simulink model "Roll_Pitch_Mixer_Disturbance_Baseline"  (R2026b)
settings: Solver=FixedStepDiscrete  StopTime=15  FixedStep=0.01
model workspace (MAT data in the model file):
  K_achieved = [1  1  1  1; -0.0742462128401  -0.0742462128401  0.0742462128401  0.0742462128401; -0.0742462128401  0.0742462128401  -0.0742462128401  0.0742462128401]
  d_arm = 0.0742462128401
undefined symbols (not defined in the file): DiscIntNeverNeededParam

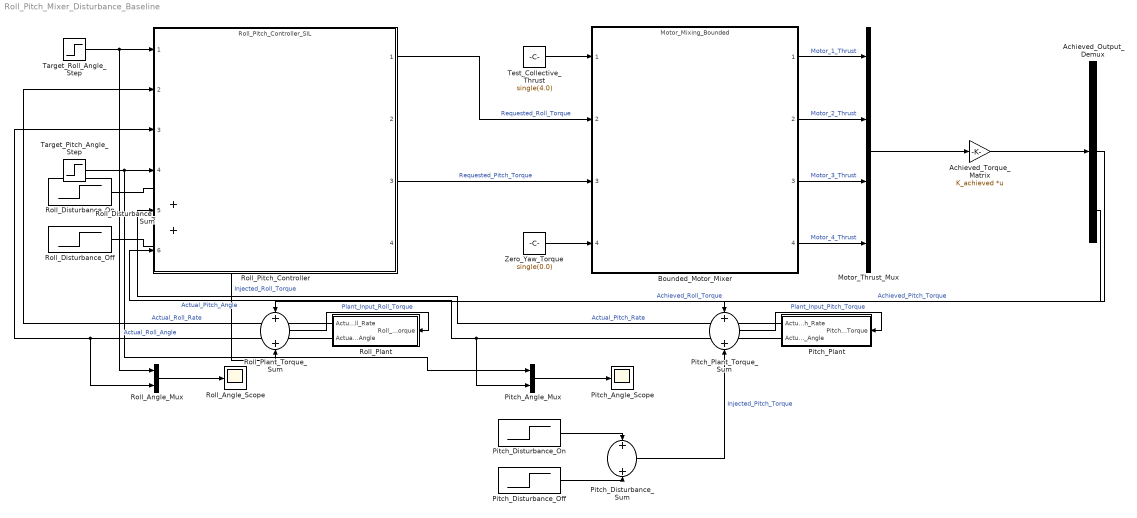
== system Roll_Pitch_Mixer_Disturbance_Baseline ==
  Achieved_Output_Demux : Demux  Outputs=3
  Achieved_Torque_Matrix : Gain  Gain=K_achieved  Multiplication=Matrix(K*u)
  Bounded_Motor_Mixer : ModelReference  ModelNameDialog=Motor_Mixing_Bounded  SimulationMode=Normal  ModelReferenceVersion=1.9
  Motor_Thrust_Mux : Mux
  Pitch_Angle_Mux : Mux  Inputs=2
  Pitch_Angle_Scope : Scope
      settings: ActiveDisplayYMinimum=-0.0589651926420629  ActiveDisplayYMaximum=0.0065516880713403208
  Pitch_Disturbance_Off : Step  Time=8  InitialValue=single(0)  FinalValue=single(0.0006)  OutDataTypeStr=single  SampleTime=0.01
  Pitch_Disturbance_On : Step  Time=7  InitialValue=single(0)  FinalValue=single(-0.0006)  OutDataTypeStr=single  SampleTime=0.01
  Pitch_Disturbance_Sum : Sum  OutDataTypeStr=single
  Pitch_Plant : Subsystem
  Pitch_Plant_Torque_Sum : Sum  OutDataTypeStr=single
  Roll_Angle_Mux : Mux  Inputs=2
  Roll_Angle_Scope : Scope
      settings: ActiveDisplayYMinimum=-0.010919480584561823  ActiveDisplayYMaximum=0.098275325261056423
  Roll_Disturbance_Off : Step  Time=8  InitialValue=single(0)  FinalValue=single(-0.001)  OutDataTypeStr=single  SampleTime=0.01
  Roll_Disturbance_On : Step  Time=7  InitialValue=single(0)  FinalValue=single(0.001)  OutDataTypeStr=single  SampleTime=0.01
  Roll_Disturbance_Sum : Sum  OutDataTypeStr=single
  Roll_Pitch_Controller : ModelReference  ModelNameDialog=Roll_Pitch_Controller_SIL  SimulationMode=Normal  ModelReferenceVersion=1.19
  Roll_Plant : Subsystem
  Roll_Plant_Torque_Sum : Sum  OutDataTypeStr=single
  Target_Pitch_Angle_Step : Step  FinalValue=-3*pi/180  OutDataTypeStr=single  SampleTime=0
  Target_Roll_Angle_Step : Step  FinalValue=5*pi/180  OutDataTypeStr=single  SampleTime=0
  Test_Collective_Thrust : Constant  Value=single(4.0)  OutDataTypeStr=single
  Zero_Yaw_Torque : Constant  Value=single(0.0)  OutDataTypeStr=single
  wires:
  Roll_Pitch_Controller/1 -> Bounded_Motor_Mixer/2  "Requested_Roll_Torque"
  Roll_Pitch_Controller/3 -> Bounded_Motor_Mixer/3  "Requested_Pitch_Torque"
  Test_Collective_Thrust/1 -> Bounded_Motor_Mixer/1
  Zero_Yaw_Torque/1 -> Bounded_Motor_Mixer/4
  Bounded_Motor_Mixer/1 -> Motor_Thrust_Mux/1  "Motor_1_Thrust"
  Bounded_Motor_Mixer/2 -> Motor_Thrust_Mux/2  "Motor_2_Thrust"
  Bounded_Motor_Mixer/3 -> Motor_Thrust_Mux/3  "Motor_3_Thrust"
  Bounded_Motor_Mixer/4 -> Motor_Thrust_Mux/4  "Motor_4_Thrust"
  Motor_Thrust_Mux/1 -> Achieved_Torque_Matrix/1
  Achieved_Torque_Matrix/1 -> Achieved_Output_Demux/1
  Roll_Plant/1(Actual_Roll_Rate) -> Roll_Pitch_Controller/2  "Actual_Roll_Rate"
  Roll_Plant/2(Actual_Roll_Angle) -> Roll_Angle_Mux/2, Roll_Pitch_Controller/3  "Actual_Roll_Angle"
  Pitch_Plant/1(Actual_Pitch_Rate) -> Roll_Pitch_Controller/5  "Actual_Pitch_Rate"
  Pitch_Plant/2(Actual_Pitch_Angle) -> Pitch_Angle_Mux/2, Roll_Pitch_Controller/6  "Actual_Pitch_Angle"
  Target_Roll_Angle_Step/1 -> Roll_Angle_Mux/1, Roll_Pitch_Controller/1
  Target_Pitch_Angle_Step/1 -> Roll_Pitch_Controller/4, Pitch_Angle_Mux/1
  Roll_Angle_Mux/1 -> Roll_Angle_Scope/1
  Pitch_Angle_Mux/1 -> Pitch_Angle_Scope/1
  Roll_Disturbance_On/1 -> Roll_Disturbance_Sum/1
  Roll_Disturbance_Off/1 -> Roll_Disturbance_Sum/2
  Achieved_Output_Demux/2 -> Roll_Plant_Torque_Sum/1  "Achieved_Roll_Torque"
  Roll_Disturbance_Sum/1 -> Roll_Plant_Torque_Sum/2  "Injected_Roll_Torque"
  Roll_Plant_Torque_Sum/1 -> Roll_Plant/1(Roll_Control_Torque)  "Plant_Input_Roll_Torque"
  Pitch_Disturbance_On/1 -> Pitch_Disturbance_Sum/1
  Pitch_Disturbance_Off/1 -> Pitch_Disturbance_Sum/2
  Achieved_Output_Demux/3 -> Pitch_Plant_Torque_Sum/1  "Achieved_Pitch_Torque"
  Pitch_Disturbance_Sum/1 -> Pitch_Plant_Torque_Sum/2  "Injected_Pitch_Torque"
  Pitch_Plant_Torque_Sum/1 -> Pitch_Plant/1(Pitch_Control_Torque)  "Plant_Input_Pitch_Torque"

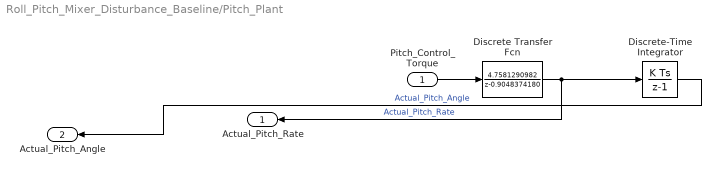
== system Roll_Pitch_Mixer_Disturbance_Baseline/Pitch_Plant ==
  Pitch_Control_Torque : Inport
  Discrete Transfer Fcn : DiscreteTransferFcn  Numerator=[0 4.7581290982]  Denominator=[1 -0.9048374180]
  Discrete-Time Integrator : DiscreteIntegrator  SampleTime=0.01  ICPrevOutput=DiscIntNeverNeededParam  ICPrevScaledInput=DiscIntNeverNeededParam
  Actual_Pitch_Rate : Outport
  Actual_Pitch_Angle : Outport  Port=2
  wires:
  Discrete Transfer Fcn/1 -> Actual_Pitch_Rate/1, Discrete-Time Integrator/1  "Actual_Pitch_Rate"
  Pitch_Control_Torque/1 -> Discrete Transfer Fcn/1
  Discrete-Time Integrator/1 -> Actual_Pitch_Angle/1  "Actual_Pitch_Angle"

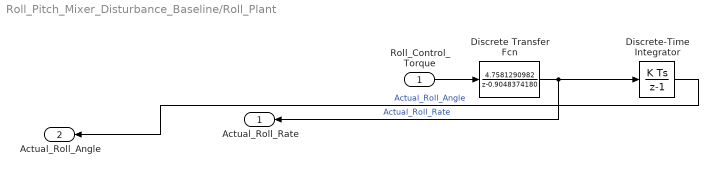
== system Roll_Pitch_Mixer_Disturbance_Baseline/Roll_Plant ==
  Roll_Control_Torque : Inport
  Discrete Transfer Fcn : DiscreteTransferFcn  Numerator=[0 4.7581290982]  Denominator=[1 -0.9048374180]
  Discrete-Time Integrator : DiscreteIntegrator  SampleTime=0.01  ICPrevOutput=DiscIntNeverNeededParam  ICPrevScaledInput=DiscIntNeverNeededParam
  Actual_Roll_Rate : Outport
  Actual_Roll_Angle : Outport  Port=2
  wires:
  Discrete-Time Integrator/1 -> Actual_Roll_Angle/1  "Actual_Roll_Angle"
  Discrete Transfer Fcn/1 -> Actual_Roll_Rate/1, Discrete-Time Integrator/1  "Actual_Roll_Rate"
  Roll_Control_Torque/1 -> Discrete Transfer Fcn/1
